simulink model "amr_step4_tracking"  (R2025a)
settings: Solver=FixedStepDiscrete  StartTime=0  StopTime=s4stopTime  FixedStep=s4dt  RelTol=1e-3
undefined symbols (not defined in the file): s4cfg, s4dt, s4env, s4ref, s4startPose
settings Model: Creator=Naresh Tuppathi  LastModifiedBy=Naresh Tuppathi
settings DataIOCC: SaveOutput=off  SignalLogging=off
settings DebuggingCC: AlgebraicLoopMsg=error  UnconnectedInputMsg=error  UnconnectedOutputMsg=error  UnconnectedLineMsg=error

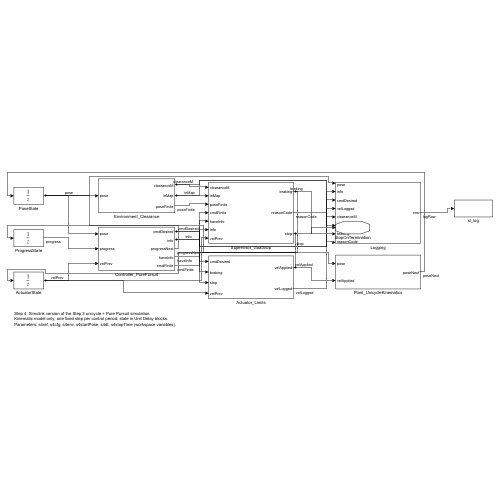
[thumbnail: Simulink's stored preview of the top-level diagram]
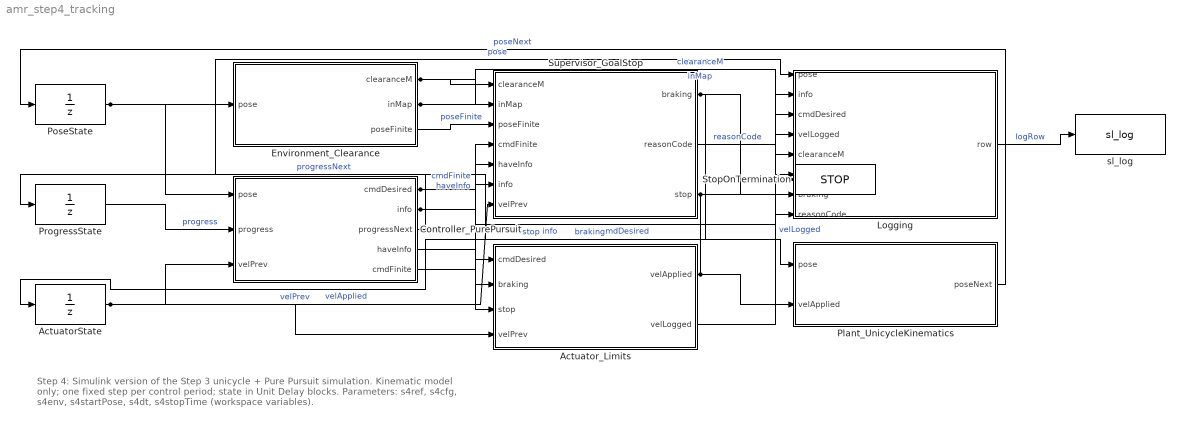
== system amr_step4_tracking ==
  note: Step 4: Simulink version of the Step 3 unicycle + Pure Pursuit simulation.
      | Kinematic model only; one fixed step per control period; state in Unit Delay blocks.
      | Parameters: s4ref, s4cfg, s4env, s4startPose, s4dt, s4stopTime (workspace variables).
  ActuatorState : UnitDelay  InitialCondition=[0; 0]  SampleTime=s4dt  HasFrameUpgradeWarning=on
  Actuator_Limits : Subsystem
  Controller_PurePursuit : Subsystem
  Environment_Clearance : Subsystem
  Logging : Subsystem
  Plant_UnicycleKinematics : Subsystem
  PoseState : UnitDelay  InitialCondition=s4startPose(:)  SampleTime=s4dt  HasFrameUpgradeWarning=on
  ProgressState : UnitDelay  SampleTime=s4dt  HasFrameUpgradeWarning=on
  StopOnTermination : Stop
  Supervisor_GoalStop : Subsystem
  sl_log : ToWorkspace  VariableName=sl_log  SampleTime=s4dt
  wires:
  PoseState/1 -> Environment_Clearance/1(pose), Controller_PurePursuit/1(pose), Plant_UnicycleKinematics/1(pose), Logging/1(pose)  "pose"
  ProgressState/1 -> Controller_PurePursuit/2(progress)  "progress"
  ActuatorState/1 -> Controller_PurePursuit/3(velPrev), Supervisor_GoalStop/7(velPrev), Actuator_Limits/4(velPrev)  "velPrev"
  Environment_Clearance/1(clearanceM) -> Supervisor_GoalStop/1(clearanceM), Logging/5(clearanceM)  "clearanceM"
  Environment_Clearance/2(inMap) -> Supervisor_GoalStop/2(inMap), Logging/6(inMap)  "inMap"
  Environment_Clearance/3(poseFinite) -> Supervisor_GoalStop/3(poseFinite)  "poseFinite"
  Controller_PurePursuit/1(cmdDesired) -> Actuator_Limits/1(cmdDesired), Logging/3(cmdDesired)  "cmdDesired"
  Controller_PurePursuit/2(info) -> Supervisor_GoalStop/6(info), Logging/2(info)  "info"
  Controller_PurePursuit/3(progressNext) -> ProgressState/1  "progressNext"
  Controller_PurePursuit/4(haveInfo) -> Supervisor_GoalStop/5(haveInfo)  "haveInfo"
  Controller_PurePursuit/5(cmdFinite) -> Supervisor_GoalStop/4(cmdFinite)  "cmdFinite"
  Supervisor_GoalStop/1(braking) -> Actuator_Limits/2(braking), Logging/7(braking)  "braking"
  Supervisor_GoalStop/2(reasonCode) -> Logging/8(reasonCode)  "reasonCode"
  Supervisor_GoalStop/3(stop) -> Actuator_Limits/3(stop), StopOnTermination/1  "stop"
  Actuator_Limits/1(velApplied) -> Plant_UnicycleKinematics/2(velApplied), ActuatorState/1  "velApplied"
  Actuator_Limits/2(velLogged) -> Logging/4(velLogged)  "velLogged"
  Plant_UnicycleKinematics/1(poseNext) -> PoseState/1  "poseNext"
  Logging/1(row) -> sl_log/1  "logRow"

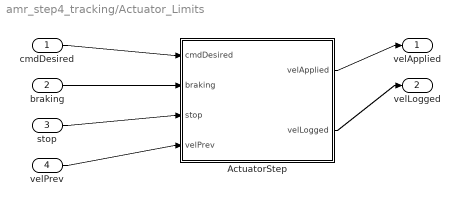
== system amr_step4_tracking/Actuator_Limits ==
  cmdDesired : Inport
  braking : Inport  Port=2
  stop : Inport  Port=3
  velPrev : Inport  Port=4
  ActuatorStep : MATLAB Function  TreatAsAtomicUnit=on
  velApplied : Outport
  velLogged : Outport  Port=2
  wires:
  cmdDesired/1 -> ActuatorStep/1(cmdDesired)
  braking/1 -> ActuatorStep/2(braking)
  stop/1 -> ActuatorStep/3(stop)
  velPrev/1 -> ActuatorStep/4(velPrev)
  ActuatorStep/1(velApplied) -> velApplied/1
  ActuatorStep/2(velLogged) -> velLogged/1

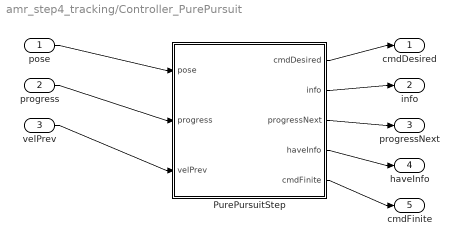
== system amr_step4_tracking/Controller_PurePursuit ==
  pose : Inport
  progress : Inport  Port=2
  velPrev : Inport  Port=3
  PurePursuitStep : MATLAB Function  TreatAsAtomicUnit=on
  cmdDesired : Outport
  info : Outport  Port=2
  progressNext : Outport  Port=3
  haveInfo : Outport  Port=4
  cmdFinite : Outport  Port=5
  wires:
  pose/1 -> PurePursuitStep/1(pose)
  progress/1 -> PurePursuitStep/2(progress)
  velPrev/1 -> PurePursuitStep/3(velPrev)
  PurePursuitStep/1(cmdDesired) -> cmdDesired/1
  PurePursuitStep/2(info) -> info/1
  PurePursuitStep/3(progressNext) -> progressNext/1
  PurePursuitStep/4(haveInfo) -> haveInfo/1
  PurePursuitStep/5(cmdFinite) -> cmdFinite/1

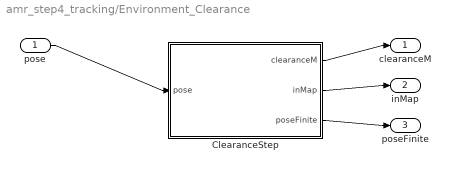
== system amr_step4_tracking/Environment_Clearance ==
  pose : Inport
  ClearanceStep : MATLAB Function  TreatAsAtomicUnit=on
  clearanceM : Outport
  inMap : Outport  Port=2
  poseFinite : Outport  Port=3
  wires:
  pose/1 -> ClearanceStep/1(pose)
  ClearanceStep/1(clearanceM) -> clearanceM/1
  ClearanceStep/2(inMap) -> inMap/1
  ClearanceStep/3(poseFinite) -> poseFinite/1

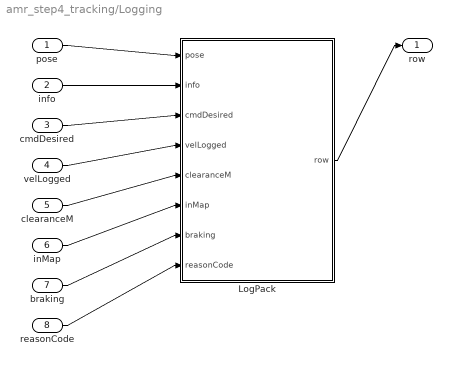
== system amr_step4_tracking/Logging ==
  pose : Inport
  info : Inport  Port=2
  cmdDesired : Inport  Port=3
  velLogged : Inport  Port=4
  clearanceM : Inport  Port=5
  inMap : Inport  Port=6
  braking : Inport  Port=7
  reasonCode : Inport  Port=8
  LogPack : MATLAB Function  TreatAsAtomicUnit=on
  row : Outport
  wires:
  pose/1 -> LogPack/1(pose)
  info/1 -> LogPack/2(info)
  cmdDesired/1 -> LogPack/3(cmdDesired)
  velLogged/1 -> LogPack/4(velLogged)
  clearanceM/1 -> LogPack/5(clearanceM)
  inMap/1 -> LogPack/6(inMap)
  braking/1 -> LogPack/7(braking)
  reasonCode/1 -> LogPack/8(reasonCode)
  LogPack/1(row) -> row/1

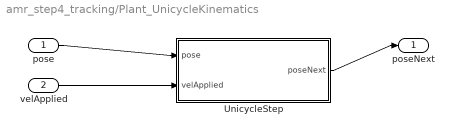
== system amr_step4_tracking/Plant_UnicycleKinematics ==
  pose : Inport
  velApplied : Inport  Port=2
  UnicycleStep : MATLAB Function  TreatAsAtomicUnit=on
  poseNext : Outport
  wires:
  pose/1 -> UnicycleStep/1(pose)
  velApplied/1 -> UnicycleStep/2(velApplied)
  UnicycleStep/1(poseNext) -> poseNext/1

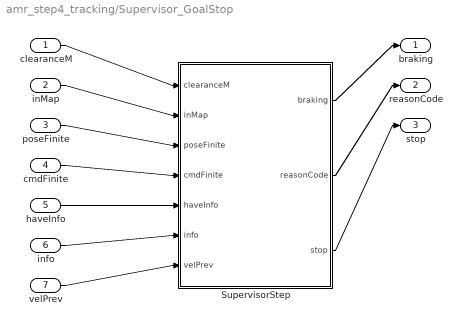
== system amr_step4_tracking/Supervisor_GoalStop ==
  clearanceM : Inport
  inMap : Inport  Port=2
  poseFinite : Inport  Port=3
  cmdFinite : Inport  Port=4
  haveInfo : Inport  Port=5
  info : Inport  Port=6
  velPrev : Inport  Port=7
  SupervisorStep : MATLAB Function  TreatAsAtomicUnit=on
  braking : Outport
  reasonCode : Outport  Port=2
  stop : Outport  Port=3
  wires:
  clearanceM/1 -> SupervisorStep/1(clearanceM)
  inMap/1 -> SupervisorStep/2(inMap)
  poseFinite/1 -> SupervisorStep/3(poseFinite)
  cmdFinite/1 -> SupervisorStep/4(cmdFinite)
  haveInfo/1 -> SupervisorStep/5(haveInfo)
  info/1 -> SupervisorStep/6(info)
  velPrev/1 -> SupervisorStep/7(velPrev)
  SupervisorStep/1(braking) -> braking/1
  SupervisorStep/2(reasonCode) -> reasonCode/1
  SupervisorStep/3(stop) -> stop/1

== matlab function amr_step4_tracking/Controller_PurePursuit/PurePursuitStep ==
  data: pose input; cmdDesired output double size=2; progress input; velPrev input; info output double size=16; progressNext output double size=1; haveInfo output double size=1; cmdFinite output double size=1; s4ref parameter; s4cfg parameter
function [cmdDesired, info, progressNext, haveInfo, cmdFinite] = fcn(pose, progress, velPrev, s4ref, s4cfg)
[cmdDesired, info, progressNext, haveInfo, cmdFinite] = slPurePursuitStep(pose, progress, velPrev, s4ref, s4cfg);
end

== matlab function amr_step4_tracking/Environment_Clearance/ClearanceStep ==
  data: pose input; clearanceM output double size=1; inMap output double size=1; poseFinite output double size=1; s4env parameter
function [clearanceM, inMap, poseFinite] = fcn(pose, s4env)
[clearanceM, inMap, poseFinite] = slClearanceStep(pose, s4env);
end

== matlab function amr_step4_tracking/Supervisor_GoalStop/SupervisorStep ==
  data: clearanceM input; braking output double size=1; inMap input; poseFinite input; cmdFinite input; haveInfo input; info input; velPrev input; reasonCode output double size=1; stop output double size=1; s4ref parameter; s4cfg parameter; s4env parameter
function [braking, reasonCode, stop] = fcn(clearanceM, inMap, poseFinite, cmdFinite, haveInfo, info, velPrev, s4ref, s4cfg, s4env)
[braking, reasonCode, stop] = slSupervisorStep(clearanceM, inMap, poseFinite, cmdFinite, haveInfo, info, velPrev, s4ref, s4cfg, s4env);
end

== matlab function amr_step4_tracking/Actuator_Limits/ActuatorStep ==
  data: cmdDesired input; velApplied output double size=2; braking input; stop input; velPrev input; velLogged output double size=2; s4cfg parameter
function [velApplied, velLogged] = fcn(cmdDesired, braking, stop, velPrev, s4cfg)
[velApplied, velLogged] = slActuatorStep(cmdDesired, braking, stop, velPrev, s4cfg);
end

== matlab function amr_step4_tracking/Plant_UnicycleKinematics/UnicycleStep ==
  data: pose input; poseNext output double size=3; velApplied input; s4cfg parameter
function poseNext  = fcn(pose, velApplied, s4cfg)
poseNext = slUnicycleStep(pose, velApplied, s4cfg);
end

== matlab function amr_step4_tracking/Logging/LogPack ==
  data: pose input; row output double size=27; info input; cmdDesired input; velLogged input; clearanceM input; inMap input; braking input; reasonCode input
function row  = fcn(pose, info, cmdDesired, velLogged, clearanceM, inMap, braking, reasonCode)
row = slLogPack(pose, info, cmdDesired, velLogged, clearanceM, inMap, braking, reasonCode);
end
